simulink model "ss2_auction_ctrl"  (R2024b)
settings: Solver=ode45  StartTime=0.0  StopTime=28800  MaxStep=1  RelTol=1e-3
undefined symbols (not defined in the file): AUC
settings Model: Creator=user  LastModifiedBy=user

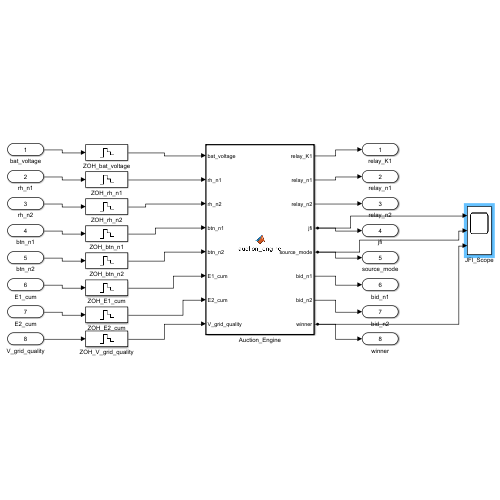
[thumbnail: Simulink's stored preview of the top-level diagram]
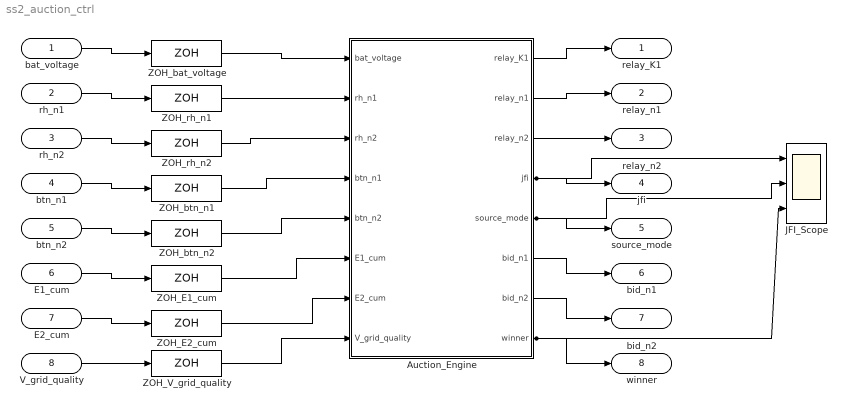
== system ss2_auction_ctrl ==
  bat_voltage : Inport
  rh_n1 : Inport  Port=2
  rh_n2 : Inport  Port=3
  btn_n1 : Inport  Port=4
  btn_n2 : Inport  Port=5
  E1_cum : Inport  Port=6
  E2_cum : Inport  Port=7
  V_grid_quality : Inport  Port=8
  Auction_Engine : MATLAB Function  TreatAsAtomicUnit=on
  JFI_Scope : Scope  NumInputPorts=3
  ZOH_E1_cum : ZeroOrderHold  SampleTime=AUC.cycle_s
  ZOH_E2_cum : ZeroOrderHold  SampleTime=AUC.cycle_s
  ZOH_V_grid_quality : ZeroOrderHold  SampleTime=AUC.cycle_s
  ZOH_bat_voltage : ZeroOrderHold  SampleTime=AUC.cycle_s
  ZOH_btn_n1 : ZeroOrderHold  SampleTime=AUC.cycle_s
  ZOH_btn_n2 : ZeroOrderHold  SampleTime=AUC.cycle_s
  ZOH_rh_n1 : ZeroOrderHold  SampleTime=AUC.cycle_s
  ZOH_rh_n2 : ZeroOrderHold  SampleTime=AUC.cycle_s
  relay_K1 : Outport
  relay_n1 : Outport  Port=2
  relay_n2 : Outport  Port=3
  jfi : Outport  Port=4
  source_mode : Outport  Port=5
  bid_n1 : Outport  Port=6
  bid_n2 : Outport  Port=7
  winner : Outport  Port=8
  wires:
  bat_voltage/1 -> ZOH_bat_voltage/1
  rh_n1/1 -> ZOH_rh_n1/1
  rh_n2/1 -> ZOH_rh_n2/1
  btn_n1/1 -> ZOH_btn_n1/1
  btn_n2/1 -> ZOH_btn_n2/1
  E1_cum/1 -> ZOH_E1_cum/1
  E2_cum/1 -> ZOH_E2_cum/1
  ZOH_bat_voltage/1 -> Auction_Engine/1(bat_voltage)
  ZOH_rh_n1/1 -> Auction_Engine/2(rh_n1)
  ZOH_rh_n2/1 -> Auction_Engine/3(rh_n2)
  ZOH_btn_n1/1 -> Auction_Engine/4(btn_n1)
  ZOH_btn_n2/1 -> Auction_Engine/5(btn_n2)
  ZOH_E1_cum/1 -> Auction_Engine/6(E1_cum)
  ZOH_E2_cum/1 -> Auction_Engine/7(E2_cum)
  Auction_Engine/1(relay_K1) -> relay_K1/1
  Auction_Engine/2(relay_n1) -> relay_n1/1
  Auction_Engine/3(relay_n2) -> relay_n2/1
  Auction_Engine/4(jfi) -> jfi/1, JFI_Scope/1
  Auction_Engine/5(source_mode) -> source_mode/1, JFI_Scope/2
  Auction_Engine/6(bid_n1) -> bid_n1/1
  Auction_Engine/7(bid_n2) -> bid_n2/1
  Auction_Engine/8(winner) -> winner/1, JFI_Scope/3
  V_grid_quality/1 -> ZOH_V_grid_quality/1
  ZOH_V_grid_quality/1 -> Auction_Engine/8(V_grid_quality)

== matlab function ss2_auction_ctrl/Auction_Engine ==
  data: bat_voltage input; relay_K1 output; rh_n1 input; rh_n2 input; btn_n1 input; btn_n2 input; E1_cum input; E2_cum input; relay_n1 output; relay_n2 output; jfi output; source_mode output; bid_n1 output; bid_n2 output; winner output; V_grid_quality input
function [relay_K1, relay_n1, relay_n2, jfi, source_mode, bid_n1, bid_n2, winner] = ...
    auction_engine(bat_voltage, rh_n1, rh_n2, btn_n1, btn_n2, E1_cum, E2_cum, V_grid_quality)
%#codegen
% AutaNet P2P Auction Protocol — Layer 2, 10-second cycle
% Decision 1: Source selection — Nigerian grid quality aware (3-state)
% Decision 2: Continuous bid function — RH maps proportionally to bid price
% Decision 3: Market clearing — highest bid wins solar
% Decision 4: JFI — Jain Fairness Index over cumulative solar energy

%% Constants
V_GRID_SW  = 11.8;   % V   battery threshold
V_LVD      = 11.6;   % V   low voltage disconnect
Q_STRONG   = 0.8;    % grid quality: strong
Q_WEAK     = 0.5;    % grid quality: weak boundary
RH_CRIT    = 0.80;   % humidity critical threshold
BID_MIN    = 100;    % bid at RH=0%
BID_CRIT   = 140;    % bid at RH=80%
BID_MAX    = 200;    % bid at RH=100%

%% Decision 1: Source selection
bat_ok      = (bat_voltage >= V_GRID_SW);
grid_strong = (V_grid_quality >= Q_STRONG);
grid_usable = (V_grid_quality >= Q_WEAK);

if bat_ok && ~grid_strong
    use_solar = true;     % grid weak — prefer solar
elseif bat_ok && grid_strong
    use_solar = true;     % both OK — prefer solar, conserve grid
elseif ~bat_ok && grid_usable
    use_solar = false;    % battery low, grid usable — protect battery
elseif ~bat_ok && ~grid_usable
    use_solar = (bat_voltage >= V_LVD);  % last resort
else
    use_solar = false;
end

%% Decision 2: Continuous bid function (piecewise linear)
% RH < 80%:  bid = 100 + (RH/0.80) x 40      → 100 to 140
% RH >= 80%: bid = 140 + ((RH-0.80)/0.20) x 60 → 140 to 200

if btn_n1 >= 0.5
    bid_n1 = BID_MAX;
elseif rh_n1 < RH_CRIT
    bid_n1 = BID_MIN + (rh_n1 / RH_CRIT) * (BID_CRIT - BID_MIN);
else
    bid_n1 = BID_CRIT + ((rh_n1 - RH_CRIT) / (1.0 - RH_CRIT)) * (BID_MAX - BID_CRIT);
end

if btn_n2 >= 0.5
    bid_n2 = BID_MAX;
elseif rh_n2 < RH_CRIT
    bid_n2 = BID_MIN + (rh_n2 / RH_CRIT) * (BID_CRIT - BID_MIN);
else
    bid_n2 = BID_CRIT + ((rh_n2 - RH_CRIT) / (1.0 - RH_CRIT)) * (BID_MAX - BID_CRIT);
end

%% Decision 3: Market clearing
if use_solar
    source_mode = 1;
    if bid_n1 >= bid_n2
        winner = 1;
    else
        winner = 2;
    end
    relay_K1 = 1;
    relay_n1 = 1;
    relay_n2 = 1;
else
    source_mode = 0;
    winner      = 0;
    relay_K1    = 0;
    relay_n1    = 1;
    relay_n2    = 1;
end

%% Decision 4: Jain Fairness Index
if E1_cum == 0 && E2_cum == 0
    jfi = 1.0;
elseif (E1_cum^2 + E2_cum^2) < 1e-9
    jfi = 1.0;
else
    jfi = (E1_cum + E2_cum)^2 / (2.0 * (E1_cum^2 + E2_cum^2));
end
jfi = min(max(jfi, 0.0), 1.0);
end
